simulink model "fixed_base_sm"  (R2025b)
settings: Solver=ode45  StartTime=0.0  StopTime=T_END  MaxStep=0.01  RelTol=1e-10  AbsTol=1e-12
values from neighbouring files (symbols this model uses):
  a0 = 1    [run_fixed_base.m]    (also in run_simscape_crosscheck.m)
  b0 = [a0/2, 0]    [run_fixed_base.m]    (also in run_simscape_crosscheck.m)
  I0 = m0*(a0^2 + a0^2)/12    (= 16.6666666667)    [run_fixed_base.m]    (also in run_simscape_crosscheck.m)
  I1 = m1*l1^2/12    (= 0.833333333333)    [run_fixed_base.m]    (also in run_simscape_crosscheck.m)
  I2 = m2*l2^2/12    (= 0.833333333333)    [run_fixed_base.m]    (also in run_simscape_crosscheck.m)
  KD = [30 10]    [run_fixed_base.m]    (also in run_simscape_crosscheck.m)
  KP = [40 20]    [run_fixed_base.m]    (also in run_simscape_crosscheck.m)
  l1 = 1    [run_fixed_base.m]    (also in run_simscape_crosscheck.m)
  l2 = 1    [run_fixed_base.m]    (also in run_simscape_crosscheck.m)
  m = modelName    [build_free_floating_sm.m]
  m0 = 100    [run_fixed_base.m]    (also in run_simscape_crosscheck.m)
  m1 = 10    [run_fixed_base.m]    (also in run_simscape_crosscheck.m)
  m2 = 10    [run_fixed_base.m]    (also in run_simscape_crosscheck.m)
  Q_GOAL = deg2rad([90 -90])    [run_fixed_base.m]    (also in run_simscape_crosscheck.m)
  Q_START = deg2rad([0 0])    [run_fixed_base.m]    (also in run_simscape_crosscheck.m)
  s = bj.child(chk{k,1}).child(chk{k,2}).series    [run_simscape_crosscheck.m]
  T_MOVE = 10    [run_fixed_base.m]    (also in run_simscape_crosscheck.m)
  Y = squeeze(out.Y_sm)    [run_fixed_base.m]    (also in run_simscape_crosscheck.m)
undefined symbols (not defined in the file or in its folder): X, Z
libraries: sm_lib x11, nesl_utility x7
settings Model: Creator=avaza  LastModifiedBy=avaza
settings DataIOCC: SaveOutput=off  TimeSaveName=t_sm  OutputOption=SpecifiedOutputTimes  OutputTimes=0:0.01:T_END
settings SimscapeCC: SimscapeLogType=all

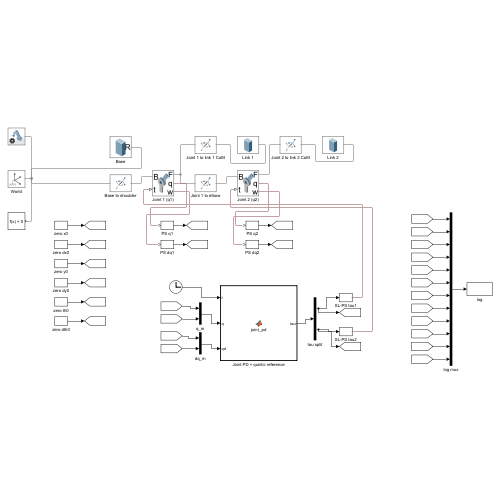
[thumbnail: Simulink's stored preview of the top-level diagram]
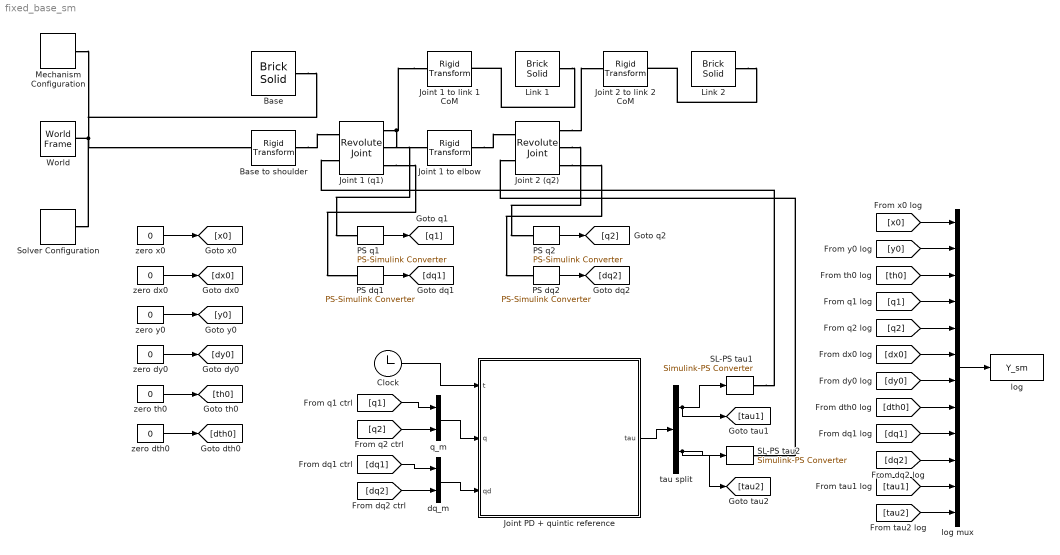
== system fixed_base_sm ==
  Base : sm_lib/Body Elements/Brick Solid  BrickDimensions=[a0 a0 0.2]  BrickDimensionsUnits=m  ExportEntireGeometry=off  InertiaType=Custom  BasedOnType=Density  Density=1000  DensityUnits=kg/m^3  Mass=m0  MassUnits=kg  CenterOfMass=[0 0 0]  CenterOfMassUnits=m  MomentsOfInertia=[0.55*I0 0.55*I0 I0]  MomentsOfInertiaUnits=kg*m^2  ProductsOfInertia=[0 0 0]  ProductsOfInertiaUnits=kg*m^2  GraphicType=FromGeometry  MarkerShape=Sphere  MarkerSize=10  GraphicVisPropType=SimpleVisualProperties  GraphicDiffuseColor=[0.6 0.6 0.7]  GraphicOpacity=1  GraphicSpecularColor=[0.5 0.5 0.5 1.0]  GraphicAmbientColor=[0.15 0.15 0.15 1.0]  GraphicEmissiveColor=[0.0 0.0 0.0 1.0]  GraphicShininess=75  DoExposeReferenceFrame=on  SerializedFrames=<Frames/>
  Base to shoulder : sm_lib/Frames and Transforms/Rigid Transform  RotationMethod=None  FollAlignAxisA=+X  BaseAlignAxisA=+Y  FollAlignAxisB=+Y  BaseAlignAxisB=+Z  RotationStandardAxis=+Z  RotationAngle=0  RotationAngleUnits=deg  RotationArbitraryAxis=[0 0 1]  RotationSequenceAxes=FollowerAxes  RotationSequence=XYX  RotationSequenceAngles=[0 0 0]  RotationSequenceAnglesUnits=deg  RotationMatrix=[1 0 0;0 1 0;0 0 1]  Quaternion=[1 0 0 0]  TranslationMethod=Cartesian  TranslationCartesianOffset=[b0(1) b0(2) 0]  TranslationCartesianOffsetUnits=m  TranslationStandardAxis=+Z  TranslationStandardOffset=0  TranslationStandardOffsetUnits=m  TranslationROffset=0  TranslationROffsetUnits=m  TranslationThetaOffset=0  TranslationThetaOffsetUnits=deg  TranslationZOffset=0  TranslationZOffsetUnits=m
  Clock : Clock
  Joint 1 (q1) : sm_lib/Joints/Revolute Joint  JointMode=Normal  CompositeWrenchDir=FollowerOnBase  CompositeWrenchFrame=BaseFrame  SenseConstraintForce=off  SenseConstraintTorque=off  SenseTotalForce=off  SenseTotalTorque=off  PositionTargetSpecify=off  PositionTargetPriority=High  PositionTargetValue=0  PositionTargetValueUnits=deg  VelocityTargetSpecify=off  VelocityTargetPriority=High  VelocityTargetValue=0  VelocityTargetValueUnits=deg/s  EquilibriumPosition=0  EquilibriumPositionUnits=deg  SpringStiffness=0  SpringStiffnessUnits=N*m/deg  DampingCoefficient=0  DampingCoefficientUnits=N*m/(deg/s)  LowerLimitSpecify=off  LowerLimitBound=-90  LowerLimitBoundUnits=deg  LowerLimitStiffness=1e4  LowerLimitStiffnessUnits=N*m/deg  LowerLimitDamping=10  LowerLimitDampingUnits=N*m/(deg/s)  LowerLimitTransitionRegionWidth=0.1  LowerLimitTransitionRegionWidthUnits=deg  UpperLimitSpecify=off  UpperLimitBound=90  UpperLimitBoundUnits=deg  UpperLimitStiffness=1e4  UpperLimitStiffnessUnits=N*m/deg  UpperLimitDamping=10  UpperLimitDampingUnits=N*m/(deg/s)  UpperLimitTransitionRegionWidth=0.1  UpperLimitTransitionRegionWidthUnits=deg  TorqueActuationMode=InputTorque  MotionActuationMode=ComputedMotion  SensePosition=on  SenseVelocity=on  SenseAcceleration=off  SenseTorqueForce=off  SenseLowerLimitTorqueForce=off  SenseUpperLimitTorqueForce=off
  Joint 1 to elbow : sm_lib/Frames and Transforms/Rigid Transform  RotationMethod=None  FollAlignAxisA=+X  BaseAlignAxisA=+Y  FollAlignAxisB=+Y  BaseAlignAxisB=+Z  RotationStandardAxis=+Z  RotationAngle=0  RotationAngleUnits=deg  RotationArbitraryAxis=[0 0 1]  RotationSequenceAxes=FollowerAxes  RotationSequence=XYX  RotationSequenceAngles=[0 0 0]  RotationSequenceAnglesUnits=deg  RotationMatrix=[1 0 0;0 1 0;0 0 1]  Quaternion=[1 0 0 0]  TranslationMethod=Cartesian  TranslationCartesianOffset=[l1 0 0]  TranslationCartesianOffsetUnits=m  TranslationStandardAxis=+Z  TranslationStandardOffset=0  TranslationStandardOffsetUnits=m  TranslationROffset=0  TranslationROffsetUnits=m  TranslationThetaOffset=0  TranslationThetaOffsetUnits=deg  TranslationZOffset=0  TranslationZOffsetUnits=m
  Joint 1 to link 1 CoM : sm_lib/Frames and Transforms/Rigid Transform  RotationMethod=None  FollAlignAxisA=+X  BaseAlignAxisA=+Y  FollAlignAxisB=+Y  BaseAlignAxisB=+Z  RotationStandardAxis=+Z  RotationAngle=0  RotationAngleUnits=deg  RotationArbitraryAxis=[0 0 1]  RotationSequenceAxes=FollowerAxes  RotationSequence=XYX  RotationSequenceAngles=[0 0 0]  RotationSequenceAnglesUnits=deg  RotationMatrix=[1 0 0;0 1 0;0 0 1]  Quaternion=[1 0 0 0]  TranslationMethod=Cartesian  TranslationCartesianOffset=[l1/2 0 0]  TranslationCartesianOffsetUnits=m  TranslationStandardAxis=+Z  TranslationStandardOffset=0  TranslationStandardOffsetUnits=m  TranslationROffset=0  TranslationROffsetUnits=m  TranslationThetaOffset=0  TranslationThetaOffsetUnits=deg  TranslationZOffset=0  TranslationZOffsetUnits=m
  Joint 2 (q2) : sm_lib/Joints/Revolute Joint  JointMode=Normal  CompositeWrenchDir=FollowerOnBase  CompositeWrenchFrame=BaseFrame  SenseConstraintForce=off  SenseConstraintTorque=off  SenseTotalForce=off  SenseTotalTorque=off  PositionTargetSpecify=off  PositionTargetPriority=High  PositionTargetValue=0  PositionTargetValueUnits=deg  VelocityTargetSpecify=off  VelocityTargetPriority=High  VelocityTargetValue=0  VelocityTargetValueUnits=deg/s  EquilibriumPosition=0  EquilibriumPositionUnits=deg  SpringStiffness=0  SpringStiffnessUnits=N*m/deg  DampingCoefficient=0  DampingCoefficientUnits=N*m/(deg/s)  LowerLimitSpecify=off  LowerLimitBound=-90  LowerLimitBoundUnits=deg  LowerLimitStiffness=1e4  LowerLimitStiffnessUnits=N*m/deg  LowerLimitDamping=10  LowerLimitDampingUnits=N*m/(deg/s)  LowerLimitTransitionRegionWidth=0.1  LowerLimitTransitionRegionWidthUnits=deg  UpperLimitSpecify=off  UpperLimitBound=90  UpperLimitBoundUnits=deg  UpperLimitStiffness=1e4  UpperLimitStiffnessUnits=N*m/deg  UpperLimitDamping=10  UpperLimitDampingUnits=N*m/(deg/s)  UpperLimitTransitionRegionWidth=0.1  UpperLimitTransitionRegionWidthUnits=deg  TorqueActuationMode=InputTorque  MotionActuationMode=ComputedMotion  SensePosition=on  SenseVelocity=on  SenseAcceleration=off  SenseTorqueForce=off  SenseLowerLimitTorqueForce=off  SenseUpperLimitTorqueForce=off
  Joint 2 to link 2 CoM : sm_lib/Frames and Transforms/Rigid Transform  RotationMethod=None  FollAlignAxisA=+X  BaseAlignAxisA=+Y  FollAlignAxisB=+Y  BaseAlignAxisB=+Z  RotationStandardAxis=+Z  RotationAngle=0  RotationAngleUnits=deg  RotationArbitraryAxis=[0 0 1]  RotationSequenceAxes=FollowerAxes  RotationSequence=XYX  RotationSequenceAngles=[0 0 0]  RotationSequenceAnglesUnits=deg  RotationMatrix=[1 0 0;0 1 0;0 0 1]  Quaternion=[1 0 0 0]  TranslationMethod=Cartesian  TranslationCartesianOffset=[l2/2 0 0]  TranslationCartesianOffsetUnits=m  TranslationStandardAxis=+Z  TranslationStandardOffset=0  TranslationStandardOffsetUnits=m  TranslationROffset=0  TranslationROffsetUnits=m  TranslationThetaOffset=0  TranslationThetaOffsetUnits=deg  TranslationZOffset=0  TranslationZOffsetUnits=m
  Joint PD + quintic reference : MATLAB Function  TreatAsAtomicUnit=on
  Link 1 : sm_lib/Body Elements/Brick Solid  BrickDimensions=[l1 0.08 0.08]  BrickDimensionsUnits=m  ExportEntireGeometry=off  InertiaType=Custom  BasedOnType=Density  Density=1000  DensityUnits=kg/m^3  Mass=m1  MassUnits=kg  CenterOfMass=[0 0 0]  CenterOfMassUnits=m  MomentsOfInertia=[0.01 I1 I1]  MomentsOfInertiaUnits=kg*m^2  ProductsOfInertia=[0 0 0]  ProductsOfInertiaUnits=kg*m^2  GraphicType=FromGeometry  MarkerShape=Sphere  MarkerSize=10  GraphicVisPropType=SimpleVisualProperties  GraphicDiffuseColor=[0.85 0.45 0.2]  GraphicOpacity=1  GraphicSpecularColor=[0.5 0.5 0.5 1.0]  GraphicAmbientColor=[0.15 0.15 0.15 1.0]  GraphicEmissiveColor=[0.0 0.0 0.0 1.0]  GraphicShininess=75  DoExposeReferenceFrame=on  SerializedFrames=<Frames/>
  Link 2 : sm_lib/Body Elements/Brick Solid  BrickDimensions=[l2 0.08 0.08]  BrickDimensionsUnits=m  ExportEntireGeometry=off  InertiaType=Custom  BasedOnType=Density  Density=1000  DensityUnits=kg/m^3  Mass=m2  MassUnits=kg  CenterOfMass=[0 0 0]  CenterOfMassUnits=m  MomentsOfInertia=[0.01 I2 I2]  MomentsOfInertiaUnits=kg*m^2  ProductsOfInertia=[0 0 0]  ProductsOfInertiaUnits=kg*m^2  GraphicType=FromGeometry  MarkerShape=Sphere  MarkerSize=10  GraphicVisPropType=SimpleVisualProperties  GraphicDiffuseColor=[0.2 0.5 0.85]  GraphicOpacity=1  GraphicSpecularColor=[0.5 0.5 0.5 1.0]  GraphicAmbientColor=[0.15 0.15 0.15 1.0]  GraphicEmissiveColor=[0.0 0.0 0.0 1.0]  GraphicShininess=75  DoExposeReferenceFrame=on  SerializedFrames=<Frames/>
  Mechanism Configuration : sm_lib/Utilities/Mechanism Configuration  UniformGravity=None  GravityVector=[0 0 -9.80665]  GravityVectorUnits=m/s^2  LinearizationDelta=0.001  JointModeTransitionNonlinearIterations=2
  PS dq1 : nesl_utility/PS-Simulink Converter  PhysicalDomain=network_engine_domain  SubClassName=ps_output  LeftPortType=input  RightPortType=output  PseudoPeriodic=off  Frequencies=[]  VectorFormat=inherit  Unit=rad/s  AffineConversion=off
  PS dq2 : nesl_utility/PS-Simulink Converter  PhysicalDomain=network_engine_domain  SubClassName=ps_output  LeftPortType=input  RightPortType=output  PseudoPeriodic=off  Frequencies=[]  VectorFormat=inherit  Unit=rad/s  AffineConversion=off
  PS q1 : nesl_utility/PS-Simulink Converter  PhysicalDomain=network_engine_domain  SubClassName=ps_output  LeftPortType=input  RightPortType=output  PseudoPeriodic=off  Frequencies=[]  VectorFormat=inherit  Unit=rad  AffineConversion=off
  PS q2 : nesl_utility/PS-Simulink Converter  PhysicalDomain=network_engine_domain  SubClassName=ps_output  LeftPortType=input  RightPortType=output  PseudoPeriodic=off  Frequencies=[]  VectorFormat=inherit  Unit=rad  AffineConversion=off
  SL-PS tau1 : nesl_utility/Simulink-PS Converter  PhysicalDomain=network_engine_domain  SubClassName=ps_input  LeftPortType=input  RightPortType=output  PseudoPeriodic=off  Frequencies=[]  NoiseDistribution=none  NoiseParameters=[]  Unit=N*m  AffineConversion=off  FilteringAndDerivatives=provide  SimscapeFilterOrder=1  InputFilterTimeConstant=0.001  UdotUserProvided=0
  SL-PS tau2 : nesl_utility/Simulink-PS Converter  PhysicalDomain=network_engine_domain  SubClassName=ps_input  LeftPortType=input  RightPortType=output  PseudoPeriodic=off  Frequencies=[]  NoiseDistribution=none  NoiseParameters=[]  Unit=N*m  AffineConversion=off  FilteringAndDerivatives=provide  SimscapeFilterOrder=1  InputFilterTimeConstant=0.001  UdotUserProvided=0
  Solver Configuration : nesl_utility/Solver Configuration  PhysicalDomain=network_engine_domain  SubClassName=solver  LeftPortType=input  RightPortType=generic  Tones=[]  Harmonics=[]  SimulateNoise=off  Profile=off  UseLocalSampling=off  EnableSwitchedLinearOptims=on  FrequencyDomain=off  UseCCode=off  RelTol=0.001  AbsTol=0.001  MinStep=1e-09  ToWorkspace=off  RevertToSquareIcSolve=off  NumHomotopyIterations=100  PhasorMode=off  PhasorModeNumHarmonics=1  ConsistencySolver=NEWTON_XTOL_AFTER_FTOL  IndexReductionMethod=DerivativeReplacement  DoDC=off  ResidualTolerance=1e-09  ConsistencyTolSource=GLOBAL  ConsistencyAbsTol=0.001  ConsistencyRelTol=0.001  ConsistencyTolFactor=0.001  UseLocalSolver=off  LocalSolverChoice=NE_BACKWARD_EULER_ADVANCER  ResolveIndetEquations=on  FunctionEvalNumThread=1  LocalSolverSampleTime=0.001  DoFixedCost=off  MaxNonlinIter=3  MaxModeIter=2  ComputeImpulses=off  ImpulseIterations=2  LinearAlgebra=auto  LinearAlgebraNumThread=0  EquationFormulation=NE_TIME_EF  DelaysMemoryBudget=1024  AutomaticFiltering=on  FilteringTimeConstant=0.001  PartitionStorageMethod=AS_NEEDED  PartitionMemoryBudget=1024  PartitionMethod=ROBUST  MultibodyUseLocalSolver=off  MultibodyLocalSolverChoice=ODE1  MultibodyLocalSolverSampleTime=0.001
  World : sm_lib/Frames and Transforms/World Frame
  dq_m : Mux  Inputs=2
  log : ToWorkspace  VariableName=Y_sm  SampleTime=-1
  log mux : Mux  Inputs=12
  q_m : Mux  Inputs=2
  tau split : Demux  Outputs=2
  zero dth0 : Constant  Value=0
  zero dx0 : Constant  Value=0
  zero dy0 : Constant  Value=0
  zero th0 : Constant  Value=0
  zero x0 : Constant  Value=0
  zero y0 : Constant  Value=0
  wires:
  zero x0/1 -> [x0]
  zero dx0/1 -> [dx0]
  zero y0/1 -> [y0]
  zero dy0/1 -> [dy0]
  zero th0/1 -> [th0]
  zero dth0/1 -> [dth0]
  PS q1/1 -> [q1]
  PS dq1/1 -> [dq1]
  PS q2/1 -> [q2]
  PS dq2/1 -> [dq2]
  [q1] -> q_m/1
  [q2] -> q_m/2
  [dq1] -> dq_m/1
  [dq2] -> dq_m/2
  Clock/1 -> Joint PD + quintic reference/1(t)
  q_m/1 -> Joint PD + quintic reference/2(q)
  dq_m/1 -> Joint PD + quintic reference/3(qd)
  Joint PD + quintic reference/1(tau) -> tau split/1
  tau split/1 -> SL-PS tau1/1, [tau1]
  tau split/2 -> SL-PS tau2/1, [tau2]
  [x0] -> log mux/1
  [y0] -> log mux/2
  [th0] -> log mux/3
  [q1] -> log mux/4
  [q2] -> log mux/5
  [dx0] -> log mux/6
  [dy0] -> log mux/7
  [dth0] -> log mux/8
  [dq1] -> log mux/9
  [dq2] -> log mux/10
  [tau1] -> log mux/11
  [tau2] -> log mux/12
  log mux/1 -> log/1
  connections:
  Mechanism Configuration/RConn1 -- Solver Configuration/RConn1 -- Base/RConn1 -- World/RConn1 -- Base to shoulder/LConn1
  Base to shoulder/RConn1 -- Joint 1 (q1)/LConn1
  Joint 1 to link 1 CoM/LConn1 -- Joint 1 (q1)/RConn1 -- Joint 1 to elbow/LConn1
  Link 1/RConn1 -- Joint 1 to link 1 CoM/RConn1
  Joint 1 to elbow/RConn1 -- Joint 2 (q2)/LConn1
  Joint 2 (q2)/RConn1 -- Joint 2 to link 2 CoM/LConn1
  Link 2/RConn1 -- Joint 2 to link 2 CoM/RConn1
  Joint 1 (q1)/RConn2 -- PS q1/LConn1
  Joint 1 (q1)/RConn3 -- PS dq1/LConn1
  Joint 2 (q2)/RConn2 -- PS q2/LConn1
  Joint 2 (q2)/RConn3 -- PS dq2/LConn1
  SL-PS tau1/RConn1 -- Joint 1 (q1)/LConn2
  SL-PS tau2/RConn1 -- Joint 2 (q2)/LConn2

== matlab function fixed_base_sm/Joint PD + quintic reference ==
  data: t input; tau output; q input; qd input; KP parameter; KD parameter; Q_START parameter; Q_GOAL parameter; T_MOVE parameter
function tau = joint_pd(t, q, qd, KP, KD, Q_START, Q_GOAL, T_MOVE)
% Quintic joint reference s = 10x^3 - 15x^4 + 6x^5 (zero vel/acc at both ends)
% and joint-space PD, exactly as simulation.py. The base is not controlled.
x = min(max(t/T_MOVE, 0), 1);
s = 10*x^3 - 15*x^4 + 6*x^5;
ds = 0;
if t < T_MOVE, ds = (30*x^2 - 60*x^3 + 30*x^4)/T_MOVE; end
q_des = Q_START(:) + s*(Q_GOAL(:) - Q_START(:));
qd_des = ds*(Q_GOAL(:) - Q_START(:));
tau = KP(:).*(q_des - q(:)) + KD(:).*(qd_des - qd(:));
